simulink model "fix_all_sync"  (R2025b)
settings: Solver=FixedStepAuto  StartTime=0.0  StopTime=10.0  FixedStep=0.001  RelTol=1e-3
values from neighbouring files (symbols this model uses):
  Dm = 1e-3    (= 0.001)    [motor_param.m]
  Jm = 0.1e-3    (= 0.0001)    [motor_param.m]
  Ld = 0.01    [motor_param.m]
  Lq = 0.02    [motor_param.m]
  p = 2    [motor_param.m]
  Phi = 0.1    [motor_param.m]
  Rs = 0.38    [motor_param.m]
libraries: fl_lib x50, nesl_utility x50, ee_lib x15, eeTransforms x10, simulink x1
(part 3 of 3)

== system fix_all_sync/Subsystem5/Plant/MechSensor ==
  Ideal Rotational Motion Sensor : fl_lib/Mechanical/Mechanical Sensors/Ideal Rotational Motion Sensor  reference=foundation.enum.MeasurementReference.difference  acceleration_port=false  velocity_port=true  position_port=true  wrap_angle=simscape.enum.onoff.off  offset=0 rad
  Ideal Torque Sensor : fl_lib/Mechanical/Mechanical Sensors/Ideal Torque Sensor
  PS-Simulink Converter : nesl_utility/PS-Simulink Converter  PhysicalDomain=network_engine_domain  SubClassName=ps_output  LeftPortType=input  RightPortType=output  PseudoPeriodic=off  Frequencies=[]  VectorFormat=1-D array  Unit=1  AffineConversion=off
  PS-Simulink Converter1 : nesl_utility/PS-Simulink Converter  PhysicalDomain=network_engine_domain  SubClassName=ps_output  LeftPortType=input  RightPortType=output  PseudoPeriodic=off  Frequencies=[]  VectorFormat=1-D array  Unit=1  AffineConversion=off
  PS-Simulink Converter2 : nesl_utility/PS-Simulink Converter  PhysicalDomain=network_engine_domain  SubClassName=ps_output  LeftPortType=input  RightPortType=output  PseudoPeriodic=off  Frequencies=[]  VectorFormat=1-D array  Unit=1  AffineConversion=off
  R1 : PMIOPort  Side=Left
  C1 : PMIOPort  Port=2  Side=Left
  R2 : PMIOPort  Port=3  Side=Right
  C2 : PMIOPort  Port=4  Side=Right
  wm : Outport  VectorParamsAs1DForOutWhenUnconnected=off
  thm : Outport  Port=2  VectorParamsAs1DForOutWhenUnconnected=off
  Tm : Outport  Port=3  VectorParamsAs1DForOutWhenUnconnected=off
  wires:
  PS-Simulink Converter/1 -> thm/1
  PS-Simulink Converter1/1 -> Tm/1
  PS-Simulink Converter2/1 -> wm/1
  connections:
  Ideal Rotational Motion Sensor/RConn3 -- PS-Simulink Converter/LConn1
  Ideal Rotational Motion Sensor/RConn1 -- C2/RConn1 -- C1/RConn1
  Ideal Torque Sensor/LConn1 -- R1/RConn1
  Ideal Torque Sensor/RConn1 -- R2/RConn1 -- Ideal Rotational Motion Sensor/LConn1
  PS-Simulink Converter1/LConn1 -- Ideal Torque Sensor/RConn2
  Ideal Rotational Motion Sensor/RConn2 -- PS-Simulink Converter2/LConn1

== system fix_all_sync/Subsystem1/Controller/DriverPeripherals/Break Algebraic Loop ==
  In1 : Inport
  Demux : Demux  Outputs=3
  Mux : Mux  Inputs=3
  Transfer Fcn : TransferFcn  Denominator=[1e-6 1]
  Transfer Fcn1 : TransferFcn  Denominator=[1e-6 1]
  Transfer Fcn2 : TransferFcn  Denominator=[1e-6 1]
  Out1 : Outport
  wires:
  In1/1 -> Demux/1
  Demux/1 -> Transfer Fcn/1
  Transfer Fcn/1 -> Mux/1
  Demux/2 -> Transfer Fcn1/1
  Transfer Fcn1/1 -> Mux/2
  Demux/3 -> Transfer Fcn2/1
  Transfer Fcn2/1 -> Mux/3
  Mux/1 -> Out1/1

== system fix_all_sync/Subsystem1/Controller/FOC/CurrentController ==
  Iqref : Inport
  Id : Inport  Port=2
  Iq : Inport  Port=3
  we : Inport  Port=4
  Integrator : Integrator
  MATLAB Function : MATLAB Function  TreatAsAtomicUnit=on
  Scope : Scope
      settings: ActiveDisplayYMinimum=-0.021972241997855933  ActiveDisplayYMaximum=0.011100987286103392  DataLoggingVariableName=ScopeData15
  Vdref : Outport  VectorParamsAs1DForOutWhenUnconnected=off
  Vqref : Outport  Port=2  VectorParamsAs1DForOutWhenUnconnected=off
  wires:
  MATLAB Function/2(Vd) -> Vdref/1
  Iqref/1 -> MATLAB Function/2(i_q_ref)
  MATLAB Function/4(e_q_bar) -> Scope/1
  we/1 -> MATLAB Function/5(we)
  Id/1 -> MATLAB Function/4(i_d)
  Iq/1 -> MATLAB Function/3(i_q)
  Integrator/1 -> MATLAB Function/1(z_q)
  MATLAB Function/1(Vq) -> Vqref/1
  MATLAB Function/3(dz_q) -> Integrator/1

== system fix_all_sync/Subsystem1/Controller/FOC/VelocityController ==
  wmref : Inport
  wm : Inport  Port=2
  Gain : Gain  Gain=1/(3/2*p*Phi)
  Integrator : Integrator
  Integrator1 : Integrator
  MATLAB Function : MATLAB Function  TreatAsAtomicUnit=on
  Iqref : Outport  VectorParamsAs1DForOutWhenUnconnected=off
  wires:
  MATLAB Function/2(dot_bar_w) -> Integrator/1
  wm/1 -> MATLAB Function/2(w_m)
  MATLAB Function/1(u_cmd) -> Gain/1
  Integrator/1 -> MATLAB Function/3(bar_w)
  Gain/1 -> Iqref/1
  wmref/1 -> MATLAB Function/1(w_ref)
  MATLAB Function/3(dot_xi) -> Integrator1/1
  Integrator1/1 -> MATLAB Function/4(xi)

== system fix_all_sync/Subsystem1/Controller/FOC/abc2dq ==
  Iabc : Inport
  thetae : Inport  Port=2
  Demux1 : Demux  Outputs=3
  Park Transform : eeTransforms/Park Transform  AxisAlignment=D-axis  PowerInvariant=off
  Terminator : Terminator
  Id : Outport  VectorParamsAs1DForOutWhenUnconnected=off
  Iq : Outport  Port=2  VectorParamsAs1DForOutWhenUnconnected=off
  wires:
  Iabc/1 -> Park Transform/1
  thetae/1 -> Park Transform/2
  Demux1/3 -> Terminator/1
  Park Transform/1 -> Demux1/1
  Demux1/1 -> Id/1
  Demux1/2 -> Iq/1

== system fix_all_sync/Subsystem1/Controller/FOC/dq2abc ==
  Vd : Inport
  Vq : Inport  Port=2
  thetae : Inport  Port=3
  Constant : Constant  Value=0
  Inverse Park Transform : eeTransforms/Inverse Park Transform  AxisAlignment=D-axis  PowerInvariant=off
  Mux : Mux  Inputs=3
  Vabc : Outport  VectorParamsAs1DForOutWhenUnconnected=off
  wires:
  thetae/1 -> Inverse Park Transform/2
  Constant/1 -> Mux/3
  Mux/1 -> Inverse Park Transform/1
  Vd/1 -> Mux/1
  Inverse Park Transform/1 -> Vabc/1
  Vq/1 -> Mux/2

== system fix_all_sync/Subsystem1/Controller/FOC/thm2the ==
  thm : Inport
  Constant : Constant  Value=2*pi
  Mod : Math  Operator=mod  SignedPower=on
  PolePairs : Gain  Gain=p
  the : Outport  VectorParamsAs1DForOutWhenUnconnected=off
  wires:
  Constant/1 -> Mod/2
  PolePairs/1 -> Mod/1
  Mod/1 -> the/1
  thm/1 -> PolePairs/1

== system fix_all_sync/Subsystem1/Controller/FOC/wm2we ==
  wm : Inport
  PolePairs : Gain  Gain=p
  we : Outport  VectorParamsAs1DForOutWhenUnconnected=off
  wires:
  wm/1 -> PolePairs/1
  PolePairs/1 -> we/1

== system fix_all_sync/Subsystem2/Controller/DriverPeripherals/Break Algebraic Loop ==
  In1 : Inport
  Demux : Demux  Outputs=3
  Mux : Mux  Inputs=3
  Transfer Fcn : TransferFcn  Denominator=[1e-6 1]
  Transfer Fcn1 : TransferFcn  Denominator=[1e-6 1]
  Transfer Fcn2 : TransferFcn  Denominator=[1e-6 1]
  Out1 : Outport
  wires:
  In1/1 -> Demux/1
  Demux/1 -> Transfer Fcn/1
  Transfer Fcn/1 -> Mux/1
  Demux/2 -> Transfer Fcn1/1
  Transfer Fcn1/1 -> Mux/2
  Demux/3 -> Transfer Fcn2/1
  Transfer Fcn2/1 -> Mux/3
  Mux/1 -> Out1/1

== system fix_all_sync/Subsystem2/Controller/FOC/CurrentController ==
  Iqref : Inport
  Id : Inport  Port=2
  Iq : Inport  Port=3
  we : Inport  Port=4
  Integrator : Integrator
  MATLAB Function : MATLAB Function  TreatAsAtomicUnit=on
  Scope : Scope
      settings: ActiveDisplayYMinimum=-0.021972241997855933  ActiveDisplayYMaximum=0.011100987286103392  DataLoggingVariableName=ScopeData8
  Vdref : Outport  VectorParamsAs1DForOutWhenUnconnected=off
  Vqref : Outport  Port=2  VectorParamsAs1DForOutWhenUnconnected=off
  wires:
  Iqref/1 -> MATLAB Function/2(i_q_ref)
  MATLAB Function/4(e_q_bar) -> Scope/1
  MATLAB Function/1(Vq) -> Vqref/1
  Integrator/1 -> MATLAB Function/1(z_q)
  MATLAB Function/2(Vd) -> Vdref/1
  MATLAB Function/3(dz_q) -> Integrator/1
  Id/1 -> MATLAB Function/4(i_d)
  we/1 -> MATLAB Function/5(we)
  Iq/1 -> MATLAB Function/3(i_q)

== system fix_all_sync/Subsystem2/Controller/FOC/VelocityController ==
  wmref : Inport
  wm : Inport  Port=2
  Gain : Gain  Gain=1/(3/2*p*Phi)
  Integrator : Integrator
  Integrator1 : Integrator
  MATLAB Function : MATLAB Function  TreatAsAtomicUnit=on
  Iqref : Outport  VectorParamsAs1DForOutWhenUnconnected=off
  wires:
  Integrator/1 -> MATLAB Function/3(bar_w)
  Integrator1/1 -> MATLAB Function/4(xi)
  wmref/1 -> MATLAB Function/1(w_ref)
  MATLAB Function/3(dot_xi) -> Integrator1/1
  MATLAB Function/1(u_cmd) -> Gain/1
  Gain/1 -> Iqref/1
  wm/1 -> MATLAB Function/2(w_m)
  MATLAB Function/2(dot_bar_w) -> Integrator/1

== system fix_all_sync/Subsystem2/Controller/FOC/abc2dq ==
  Iabc : Inport
  thetae : Inport  Port=2
  Demux1 : Demux  Outputs=3
  Park Transform : eeTransforms/Park Transform  AxisAlignment=D-axis  PowerInvariant=off
  Terminator : Terminator
  Id : Outport  VectorParamsAs1DForOutWhenUnconnected=off
  Iq : Outport  Port=2  VectorParamsAs1DForOutWhenUnconnected=off
  wires:
  Iabc/1 -> Park Transform/1
  thetae/1 -> Park Transform/2
  Demux1/3 -> Terminator/1
  Park Transform/1 -> Demux1/1
  Demux1/1 -> Id/1
  Demux1/2 -> Iq/1

== system fix_all_sync/Subsystem2/Controller/FOC/dq2abc ==
  Vd : Inport
  Vq : Inport  Port=2
  thetae : Inport  Port=3
  Constant : Constant  Value=0
  Inverse Park Transform : eeTransforms/Inverse Park Transform  AxisAlignment=D-axis  PowerInvariant=off
  Mux : Mux  Inputs=3
  Vabc : Outport  VectorParamsAs1DForOutWhenUnconnected=off
  wires:
  thetae/1 -> Inverse Park Transform/2
  Constant/1 -> Mux/3
  Mux/1 -> Inverse Park Transform/1
  Vd/1 -> Mux/1
  Inverse Park Transform/1 -> Vabc/1
  Vq/1 -> Mux/2

== system fix_all_sync/Subsystem2/Controller/FOC/thm2the ==
  thm : Inport
  Constant : Constant  Value=2*pi
  Mod : Math  Operator=mod  SignedPower=on
  PolePairs : Gain  Gain=p
  the : Outport  VectorParamsAs1DForOutWhenUnconnected=off
  wires:
  Constant/1 -> Mod/2
  PolePairs/1 -> Mod/1
  Mod/1 -> the/1
  thm/1 -> PolePairs/1

== system fix_all_sync/Subsystem2/Controller/FOC/wm2we ==
  wm : Inport
  PolePairs : Gain  Gain=p
  we : Outport  VectorParamsAs1DForOutWhenUnconnected=off
  wires:
  wm/1 -> PolePairs/1
  PolePairs/1 -> we/1

== system fix_all_sync/Subsystem3/Controller/DriverPeripherals/Break Algebraic Loop ==
  In1 : Inport
  Demux : Demux  Outputs=3
  Mux : Mux  Inputs=3
  Transfer Fcn : TransferFcn  Denominator=[1e-6 1]
  Transfer Fcn1 : TransferFcn  Denominator=[1e-6 1]
  Transfer Fcn2 : TransferFcn  Denominator=[1e-6 1]
  Out1 : Outport
  wires:
  In1/1 -> Demux/1
  Demux/1 -> Transfer Fcn/1
  Transfer Fcn/1 -> Mux/1
  Demux/2 -> Transfer Fcn1/1
  Transfer Fcn1/1 -> Mux/2
  Demux/3 -> Transfer Fcn2/1
  Transfer Fcn2/1 -> Mux/3
  Mux/1 -> Out1/1

== system fix_all_sync/Subsystem3/Controller/FOC/CurrentController ==
  Iqref : Inport
  Id : Inport  Port=2
  Iq : Inport  Port=3
  we : Inport  Port=4
  Integrator : Integrator
  MATLAB Function : MATLAB Function  TreatAsAtomicUnit=on
  Scope : Scope
      settings: ActiveDisplayYMinimum=-0.021972241997855933  ActiveDisplayYMaximum=0.011100987286103392  DataLoggingVariableName=ScopeData9
  Vdref : Outport  VectorParamsAs1DForOutWhenUnconnected=off
  Vqref : Outport  Port=2  VectorParamsAs1DForOutWhenUnconnected=off
  wires:
  Iqref/1 -> MATLAB Function/2(i_q_ref)
  MATLAB Function/4(e_q_bar) -> Scope/1
  MATLAB Function/1(Vq) -> Vqref/1
  Integrator/1 -> MATLAB Function/1(z_q)
  MATLAB Function/2(Vd) -> Vdref/1
  MATLAB Function/3(dz_q) -> Integrator/1
  Id/1 -> MATLAB Function/4(i_d)
  Iq/1 -> MATLAB Function/3(i_q)
  we/1 -> MATLAB Function/5(we)

== system fix_all_sync/Subsystem3/Controller/FOC/VelocityController ==
  wmref : Inport
  wm : Inport  Port=2
  Gain : Gain  Gain=1/(3/2*p*Phi)
  Integrator : Integrator
  Integrator1 : Integrator
  MATLAB Function : MATLAB Function  TreatAsAtomicUnit=on
  Iqref : Outport  VectorParamsAs1DForOutWhenUnconnected=off
  wires:
  Integrator/1 -> MATLAB Function/3(bar_w)
  Integrator1/1 -> MATLAB Function/4(xi)
  wmref/1 -> MATLAB Function/1(w_ref)
  MATLAB Function/3(dot_xi) -> Integrator1/1
  MATLAB Function/1(u_cmd) -> Gain/1
  Gain/1 -> Iqref/1
  wm/1 -> MATLAB Function/2(w_m)
  MATLAB Function/2(dot_bar_w) -> Integrator/1

== system fix_all_sync/Subsystem3/Controller/FOC/abc2dq ==
  Iabc : Inport
  thetae : Inport  Port=2
  Demux1 : Demux  Outputs=3
  Park Transform : eeTransforms/Park Transform  AxisAlignment=D-axis  PowerInvariant=off
  Terminator : Terminator
  Id : Outport  VectorParamsAs1DForOutWhenUnconnected=off
  Iq : Outport  Port=2  VectorParamsAs1DForOutWhenUnconnected=off
  wires:
  Iabc/1 -> Park Transform/1
  thetae/1 -> Park Transform/2
  Demux1/3 -> Terminator/1
  Park Transform/1 -> Demux1/1
  Demux1/1 -> Id/1
  Demux1/2 -> Iq/1

== system fix_all_sync/Subsystem3/Controller/FOC/dq2abc ==
  Vd : Inport
  Vq : Inport  Port=2
  thetae : Inport  Port=3
  Constant : Constant  Value=0
  Inverse Park Transform : eeTransforms/Inverse Park Transform  AxisAlignment=D-axis  PowerInvariant=off
  Mux : Mux  Inputs=3
  Vabc : Outport  VectorParamsAs1DForOutWhenUnconnected=off
  wires:
  thetae/1 -> Inverse Park Transform/2
  Constant/1 -> Mux/3
  Mux/1 -> Inverse Park Transform/1
  Vd/1 -> Mux/1
  Inverse Park Transform/1 -> Vabc/1
  Vq/1 -> Mux/2

== system fix_all_sync/Subsystem3/Controller/FOC/thm2the ==
  thm : Inport
  Constant : Constant  Value=2*pi
  Mod : Math  Operator=mod  SignedPower=on
  PolePairs : Gain  Gain=p
  the : Outport  VectorParamsAs1DForOutWhenUnconnected=off
  wires:
  Constant/1 -> Mod/2
  PolePairs/1 -> Mod/1
  Mod/1 -> the/1
  thm/1 -> PolePairs/1

== system fix_all_sync/Subsystem3/Controller/FOC/wm2we ==
  wm : Inport
  PolePairs : Gain  Gain=p
  we : Outport  VectorParamsAs1DForOutWhenUnconnected=off
  wires:
  wm/1 -> PolePairs/1
  PolePairs/1 -> we/1

== system fix_all_sync/Subsystem4/Controller/DriverPeripherals/Break Algebraic Loop ==
  In1 : Inport
  Demux : Demux  Outputs=3
  Mux : Mux  Inputs=3
  Transfer Fcn : TransferFcn  Denominator=[1e-6 1]
  Transfer Fcn1 : TransferFcn  Denominator=[1e-6 1]
  Transfer Fcn2 : TransferFcn  Denominator=[1e-6 1]
  Out1 : Outport
  wires:
  In1/1 -> Demux/1
  Demux/1 -> Transfer Fcn/1
  Transfer Fcn/1 -> Mux/1
  Demux/2 -> Transfer Fcn1/1
  Transfer Fcn1/1 -> Mux/2
  Demux/3 -> Transfer Fcn2/1
  Transfer Fcn2/1 -> Mux/3
  Mux/1 -> Out1/1

== system fix_all_sync/Subsystem4/Controller/FOC/CurrentController ==
  Iqref : Inport
  Id : Inport  Port=2
  Iq : Inport  Port=3
  we : Inport  Port=4
  Integrator : Integrator
  MATLAB Function : MATLAB Function  TreatAsAtomicUnit=on
  Scope : Scope
      settings: ActiveDisplayYMinimum=-0.021972241997855933  ActiveDisplayYMaximum=0.011100987286103392  DataLoggingVariableName=ScopeData10
  Vdref : Outport  VectorParamsAs1DForOutWhenUnconnected=off
  Vqref : Outport  Port=2  VectorParamsAs1DForOutWhenUnconnected=off
  wires:
  Iqref/1 -> MATLAB Function/2(i_q_ref)
  MATLAB Function/4(e_q_bar) -> Scope/1
  MATLAB Function/1(Vq) -> Vqref/1
  Integrator/1 -> MATLAB Function/1(z_q)
  MATLAB Function/2(Vd) -> Vdref/1
  MATLAB Function/3(dz_q) -> Integrator/1
  Id/1 -> MATLAB Function/4(i_d)
  Iq/1 -> MATLAB Function/3(i_q)
  we/1 -> MATLAB Function/5(we)

== system fix_all_sync/Subsystem4/Controller/FOC/VelocityController ==
  wmref : Inport
  wm : Inport  Port=2
  Gain : Gain  Gain=1/(3/2*p*Phi)
  Integrator : Integrator
  Integrator1 : Integrator
  MATLAB Function : MATLAB Function  TreatAsAtomicUnit=on
  Iqref : Outport  VectorParamsAs1DForOutWhenUnconnected=off
  wires:
  Integrator/1 -> MATLAB Function/3(bar_w)
  Integrator1/1 -> MATLAB Function/4(xi)
  wmref/1 -> MATLAB Function/1(w_ref)
  MATLAB Function/3(dot_xi) -> Integrator1/1
  MATLAB Function/1(u_cmd) -> Gain/1
  Gain/1 -> Iqref/1
  wm/1 -> MATLAB Function/2(w_m)
  MATLAB Function/2(dot_bar_w) -> Integrator/1

== system fix_all_sync/Subsystem4/Controller/FOC/abc2dq ==
  Iabc : Inport
  thetae : Inport  Port=2
  Demux1 : Demux  Outputs=3
  Park Transform : eeTransforms/Park Transform  AxisAlignment=D-axis  PowerInvariant=off
  Terminator : Terminator
  Id : Outport  VectorParamsAs1DForOutWhenUnconnected=off
  Iq : Outport  Port=2  VectorParamsAs1DForOutWhenUnconnected=off
  wires:
  Iabc/1 -> Park Transform/1
  thetae/1 -> Park Transform/2
  Demux1/3 -> Terminator/1
  Park Transform/1 -> Demux1/1
  Demux1/1 -> Id/1
  Demux1/2 -> Iq/1

== system fix_all_sync/Subsystem4/Controller/FOC/dq2abc ==
  Vd : Inport
  Vq : Inport  Port=2
  thetae : Inport  Port=3
  Constant : Constant  Value=0
  Inverse Park Transform : eeTransforms/Inverse Park Transform  AxisAlignment=D-axis  PowerInvariant=off
  Mux : Mux  Inputs=3
  Vabc : Outport  VectorParamsAs1DForOutWhenUnconnected=off
  wires:
  thetae/1 -> Inverse Park Transform/2
  Constant/1 -> Mux/3
  Mux/1 -> Inverse Park Transform/1
  Vd/1 -> Mux/1
  Inverse Park Transform/1 -> Vabc/1
  Vq/1 -> Mux/2

== system fix_all_sync/Subsystem4/Controller/FOC/thm2the ==
  thm : Inport
  Constant : Constant  Value=2*pi
  Mod : Math  Operator=mod  SignedPower=on
  PolePairs : Gain  Gain=p
  the : Outport  VectorParamsAs1DForOutWhenUnconnected=off
  wires:
  Constant/1 -> Mod/2
  PolePairs/1 -> Mod/1
  Mod/1 -> the/1
  thm/1 -> PolePairs/1

== system fix_all_sync/Subsystem4/Controller/FOC/wm2we ==
  wm : Inport
  PolePairs : Gain  Gain=p
  we : Outport  VectorParamsAs1DForOutWhenUnconnected=off
  wires:
  wm/1 -> PolePairs/1
  PolePairs/1 -> we/1

== system fix_all_sync/Subsystem5/Controller/DriverPeripherals/Break Algebraic Loop ==
  In1 : Inport
  Demux : Demux  Outputs=3
  Mux : Mux  Inputs=3
  Transfer Fcn : TransferFcn  Denominator=[1e-6 1]
  Transfer Fcn1 : TransferFcn  Denominator=[1e-6 1]
  Transfer Fcn2 : TransferFcn  Denominator=[1e-6 1]
  Out1 : Outport
  wires:
  In1/1 -> Demux/1
  Demux/1 -> Transfer Fcn/1
  Transfer Fcn/1 -> Mux/1
  Demux/2 -> Transfer Fcn1/1
  Transfer Fcn1/1 -> Mux/2
  Demux/3 -> Transfer Fcn2/1
  Transfer Fcn2/1 -> Mux/3
  Mux/1 -> Out1/1

== system fix_all_sync/Subsystem5/Controller/FOC/CurrentController ==
  Iqref : Inport
  Id : Inport  Port=2
  Iq : Inport  Port=3
  we : Inport  Port=4
  Integrator : Integrator
  MATLAB Function : MATLAB Function  TreatAsAtomicUnit=on
  Scope : Scope
      settings: ActiveDisplayYMinimum=-0.021972241997855933  ActiveDisplayYMaximum=0.011100987286103392  DataLoggingVariableName=ScopeData11
  Vdref : Outport  VectorParamsAs1DForOutWhenUnconnected=off
  Vqref : Outport  Port=2  VectorParamsAs1DForOutWhenUnconnected=off
  wires:
  Iqref/1 -> MATLAB Function/2(i_q_ref)
  MATLAB Function/4(e_q_bar) -> Scope/1
  MATLAB Function/1(Vq) -> Vqref/1
  Integrator/1 -> MATLAB Function/1(z_q)
  MATLAB Function/2(Vd) -> Vdref/1
  MATLAB Function/3(dz_q) -> Integrator/1
  Id/1 -> MATLAB Function/4(i_d)
  Iq/1 -> MATLAB Function/3(i_q)
  we/1 -> MATLAB Function/5(we)

== system fix_all_sync/Subsystem5/Controller/FOC/VelocityController ==
  wmref : Inport
  wm : Inport  Port=2
  Gain : Gain  Gain=1/(3/2*p*Phi)
  Integrator : Integrator
  Integrator1 : Integrator
  MATLAB Function : MATLAB Function  TreatAsAtomicUnit=on
  Iqref : Outport  VectorParamsAs1DForOutWhenUnconnected=off
  wires:
  Integrator/1 -> MATLAB Function/3(bar_w)
  Integrator1/1 -> MATLAB Function/4(xi)
  wmref/1 -> MATLAB Function/1(w_ref)
  MATLAB Function/3(dot_xi) -> Integrator1/1
  MATLAB Function/1(u_cmd) -> Gain/1
  Gain/1 -> Iqref/1
  wm/1 -> MATLAB Function/2(w_m)
  MATLAB Function/2(dot_bar_w) -> Integrator/1

== system fix_all_sync/Subsystem5/Controller/FOC/abc2dq ==
  Iabc : Inport
  thetae : Inport  Port=2
  Demux1 : Demux  Outputs=3
  Park Transform : eeTransforms/Park Transform  AxisAlignment=D-axis  PowerInvariant=off
  Terminator : Terminator
  Id : Outport  VectorParamsAs1DForOutWhenUnconnected=off
  Iq : Outport  Port=2  VectorParamsAs1DForOutWhenUnconnected=off
  wires:
  Iabc/1 -> Park Transform/1
  thetae/1 -> Park Transform/2
  Demux1/3 -> Terminator/1
  Park Transform/1 -> Demux1/1
  Demux1/1 -> Id/1
  Demux1/2 -> Iq/1

== system fix_all_sync/Subsystem5/Controller/FOC/dq2abc ==
  Vd : Inport
  Vq : Inport  Port=2
  thetae : Inport  Port=3
  Constant : Constant  Value=0
  Inverse Park Transform : eeTransforms/Inverse Park Transform  AxisAlignment=D-axis  PowerInvariant=off
  Mux : Mux  Inputs=3
  Vabc : Outport  VectorParamsAs1DForOutWhenUnconnected=off
  wires:
  thetae/1 -> Inverse Park Transform/2
  Constant/1 -> Mux/3
  Mux/1 -> Inverse Park Transform/1
  Vd/1 -> Mux/1
  Inverse Park Transform/1 -> Vabc/1
  Vq/1 -> Mux/2

== system fix_all_sync/Subsystem5/Controller/FOC/thm2the ==
  thm : Inport
  Constant : Constant  Value=2*pi
  Mod : Math  Operator=mod  SignedPower=on
  PolePairs : Gain  Gain=p
  the : Outport  VectorParamsAs1DForOutWhenUnconnected=off
  wires:
  Constant/1 -> Mod/2
  PolePairs/1 -> Mod/1
  Mod/1 -> the/1
  thm/1 -> PolePairs/1

== system fix_all_sync/Subsystem5/Controller/FOC/wm2we ==
  wm : Inport
  PolePairs : Gain  Gain=p
  we : Outport  VectorParamsAs1DForOutWhenUnconnected=off
  wires:
  wm/1 -> PolePairs/1
  PolePairs/1 -> we/1

== matlab function fix_all_sync/Subsystem2/Controller/FOC/VelocityController/MATLAB Function ==
  data: w_ref input; u_cmd output; w_m input; bar_w input; xi input; Jm parameter; Dm parameter; dot_bar_w output; dot_xi output
function [u_cmd, dot_bar_w, dot_xi] = FixedTimeController(w_ref, w_m, bar_w, xi, Jm, Dm)

    lambda1  = 5;   lambda2 = 5;   lambda3 = 6;
    tau      = 0.5; vartheta = 1.5;
    k_w = 6; k1 = 5; k2 = 5;

    k_i = 20;

    kappa0 = 30;     % 线性积分增益（新增，压制小误差）
    kappa1 = 20;     % 固定时间项增益
    kappa2 = 20;
    alpha1 = 0.5;
    alpha2 = 1.5;

    pow_func = @(x, gamma) abs(x)^gamma * sign(x);

    % 公式(117) 滤波器
    e_w = bar_w - w_ref;
    dot_bar_w = (1/tau) * ( -lambda1 * pow_func(e_w, 0.5) ...
                            -lambda2 * pow_func(e_w, vartheta) ...
                            -lambda3 * e_w );

    s   = w_m - bar_w;
    e_v = w_m - w_ref;

    % 混合固定时间积分
    dot_xi = kappa0 * e_v ...
           + kappa1 * pow_func(e_v, alpha1) ...
           + kappa2 * pow_func(e_v, alpha2);

    TL_hat_int = k_i * xi;

    feedback = -k_w * s ...
               - k1 * pow_func(s, 0.5) ...
               - k2 * pow_func(s, vartheta);

    u_cmd = Jm * dot_bar_w + Dm * bar_w - TL_hat_int + feedback;
end

== matlab function fix_all_sync/Subsystem3/Controller/FOC/VelocityController/MATLAB Function ==
  data: w_ref input; u_cmd output; w_m input; bar_w input; xi input; Jm parameter; Dm parameter; dot_bar_w output; dot_xi output
function [u_cmd, dot_bar_w, dot_xi] = FixedTimeController(w_ref, w_m, bar_w, xi, Jm, Dm)

    lambda1  = 5;   lambda2 = 5;   lambda3 = 6;
    tau      = 0.5; vartheta = 1.5;
    k_w = 6; k1 = 5; k2 = 5;

    k_i = 20;

    kappa0 = 30;     % 线性积分增益（新增，压制小误差）
    kappa1 = 20;     % 固定时间项增益
    kappa2 = 20;
    alpha1 = 0.5;
    alpha2 = 1.5;

    pow_func = @(x, gamma) abs(x)^gamma * sign(x);

    % 公式(117) 滤波器
    e_w = bar_w - w_ref;
    dot_bar_w = (1/tau) * ( -lambda1 * pow_func(e_w, 0.5) ...
                            -lambda2 * pow_func(e_w, vartheta) ...
                            -lambda3 * e_w );

    s   = w_m - bar_w;
    e_v = w_m - w_ref;

    % 混合固定时间积分
    dot_xi = kappa0 * e_v ...
           + kappa1 * pow_func(e_v, alpha1) ...
           + kappa2 * pow_func(e_v, alpha2);

    TL_hat_int = k_i * xi;

    feedback = -k_w * s ...
               - k1 * pow_func(s, 0.5) ...
               - k2 * pow_func(s, vartheta);

    u_cmd = Jm * dot_bar_w + Dm * bar_w - TL_hat_int + feedback;
end

== matlab function fix_all_sync/Subsystem4/Controller/FOC/VelocityController/MATLAB Function ==
  data: w_ref input; u_cmd output; w_m input; bar_w input; xi input; Jm parameter; Dm parameter; dot_bar_w output; dot_xi output
function [u_cmd, dot_bar_w, dot_xi] = FixedTimeController(w_ref, w_m, bar_w, xi, Jm, Dm)

    lambda1  = 5;   lambda2 = 5;   lambda3 = 6;
    tau      = 0.5; vartheta = 1.5;
    k_w = 6; k1 = 5; k2 = 5;

    k_i = 20;

    kappa0 = 30;     % 线性积分增益（新增，压制小误差）
    kappa1 = 20;     % 固定时间项增益
    kappa2 = 20;
    alpha1 = 0.5;
    alpha2 = 1.5;

    pow_func = @(x, gamma) abs(x)^gamma * sign(x);

    % 公式(117) 滤波器
    e_w = bar_w - w_ref;
    dot_bar_w = (1/tau) * ( -lambda1 * pow_func(e_w, 0.5) ...
                            -lambda2 * pow_func(e_w, vartheta) ...
                            -lambda3 * e_w );

    s   = w_m - bar_w;
    e_v = w_m - w_ref;

    % 混合固定时间积分
    dot_xi = kappa0 * e_v ...
           + kappa1 * pow_func(e_v, alpha1) ...
           + kappa2 * pow_func(e_v, alpha2);

    TL_hat_int = k_i * xi;

    feedback = -k_w * s ...
               - k1 * pow_func(s, 0.5) ...
               - k2 * pow_func(s, vartheta);

    u_cmd = Jm * dot_bar_w + Dm * bar_w - TL_hat_int + feedback;
end

== matlab function fix_all_sync/Subsystem5/Controller/FOC/VelocityController/MATLAB Function ==
  data: w_ref input; u_cmd output; w_m input; bar_w input; xi input; Jm parameter; Dm parameter; dot_bar_w output; dot_xi output
function [u_cmd, dot_bar_w, dot_xi] = FixedTimeController(w_ref, w_m, bar_w, xi, Jm, Dm)

    lambda1  = 5;   lambda2 = 5;   lambda3 = 6;
    tau      = 0.5; vartheta = 1.5;
    k_w = 6; k1 = 5; k2 = 5;

    k_i = 20;

    kappa0 = 30;     % 线性积分增益（新增，压制小误差）
    kappa1 = 20;     % 固定时间项增益
    kappa2 = 20;
    alpha1 = 0.5;
    alpha2 = 1.5;

    pow_func = @(x, gamma) abs(x)^gamma * sign(x);

    % 公式(117) 滤波器
    e_w = bar_w - w_ref;
    dot_bar_w = (1/tau) * ( -lambda1 * pow_func(e_w, 0.5) ...
                            -lambda2 * pow_func(e_w, vartheta) ...
                            -lambda3 * e_w );

    s   = w_m - bar_w;
    e_v = w_m - w_ref;

    % 混合固定时间积分
    dot_xi = kappa0 * e_v ...
           + kappa1 * pow_func(e_v, alpha1) ...
           + kappa2 * pow_func(e_v, alpha2);

    TL_hat_int = k_i * xi;

    feedback = -k_w * s ...
               - k1 * pow_func(s, 0.5) ...
               - k2 * pow_func(s, vartheta);

    u_cmd = Jm * dot_bar_w + Dm * bar_w - TL_hat_int + feedback;
end

== matlab function fix_all_sync/Subsystem7/MATLAB Function4 ==
  data: dth_hat output; dom_hat output; theta0 input; th_hat input; om_hat input
%% ObserverRHS
function [dth_hat, dom_hat] = ObserverRHS(theta0, th_hat, om_hat)
%#codegen
n = 5;
L = 2*eye(n) - diag(ones(n-1,1),1) - diag(ones(n-1,1),-1);
B = diag([1, 0, 1, 0, 0]);

a1 = 0.7;  a2 = 1.3;
a3 = 2*a1-1;  a4 = 2*a2-1;
c1 = 50;  c2 = 50;     % ★ 加大
c3 = 500; c4 = 500;    % ★ 加大

sig = @(x,a) sign(x).*abs(x).^a;

th0 = theta0(1);       % ★ 强制标量

e = zeros(n,1);
for i = 1:n
    ei = 0;
    for j = 1:n
        if i ~= j && L(i,j) ~= 0
            ei = ei + (-L(i,j))*(th_hat(i) - th_hat(j));
        end
    end
    if B(i,i) == 1
        ei = ei + (th_hat(i) - th0);
    end
    e(i) = ei;
end

dth_hat = om_hat - c1*sig(e,a1) - c2*sig(e,a2);
dom_hat =          - c3*sig(e,a3) - c4*sig(e,a4);
end

== matlab function fix_all_sync/Subsystem1/Controller/FOC/CurrentController/MATLAB Function ==
  data: z_q input; Vq output; i_q_ref input; i_q input; i_d input; we input; Vd output; dz_q output; e_q_bar output; Rs parameter; Ld parameter; Lq parameter; Phi parameter
function [Vq, Vd, dz_q, e_q_bar] = smc_ctrl(z_q, i_q_ref, i_q, i_d, we, Rs, Ld, Lq, Phi)
%#codegen
% ============================================================
%  PMSM 超螺旋滑模电流控制器
%  Rs, Ld, Lq, Phi, p 及滑模增益均由 Parameter 作用域提供
% ============================================================

%% ---------- 滑模参数 (仍然写死, 因为它们只属于控制器) ----------
r1  = 0.5;   r2  = 1.5;
rho1 = 0.5;  rho2 = 1.5;

k_q1 = -500;  k_q2 = -400;
k_d1 = -500;  k_d2 = -400;

lam_q1 = 50;   lam_q2 = 50;

%% ---------- 滑模面 ----------
e_q_bar = i_q - z_q;

%% ---------- 迭代部分的导数 (积分交给 Simulink) ----------
e_z  = z_q - i_q_ref;
dz_q = -lam_q1 * sig(e_z, rho1) - lam_q2 * sig(e_z, rho2);

%% ---------- u_q (非迭代) ----------
Vq = Lq * ( dz_q ...
             + k_q1 * sig(e_q_bar, r1) ...
             + k_q2 * sig(e_q_bar, r2) ) ...
      + Rs * z_q ...
      + Ld * we * i_d ...
      + we * Phi ;

%% ---------- u_d (非迭代) ----------
Vd = Ld * ( k_d1 * sig(i_d, r1) ...
             + k_d2 * sig(i_d, r2) ) ...
      + Rs * i_d ...
      + Lq * we * i_q;

end

function y = sig(x, r)
    y = abs(x)^r * sign(x);
end

== matlab function fix_all_sync/Subsystem1/Controller/FOC/VelocityController/MATLAB Function ==
  data: w_ref input; u_cmd output; w_m input; bar_w input; xi input; Jm parameter; Dm parameter; dot_bar_w output; dot_xi output
function [u_cmd, dot_bar_w, dot_xi] = FixedTimeController(w_ref, w_m, bar_w, xi, Jm, Dm)

    lambda1  = 5;   lambda2 = 5;   lambda3 = 6;
    tau      = 0.5; vartheta = 1.5;
    k_w = 6; k1 = 5; k2 = 5;

    k_i = 20;

    kappa0 = 30;     % 线性积分增益（新增，压制小误差）
    kappa1 = 20;     % 固定时间项增益
    kappa2 = 20;
    alpha1 = 0.5;
    alpha2 = 1.5;

    pow_func = @(x, gamma) abs(x)^gamma * sign(x);

    % 公式(117) 滤波器
    e_w = bar_w - w_ref;
    dot_bar_w = (1/tau) * ( -lambda1 * pow_func(e_w, 0.5) ...
                            -lambda2 * pow_func(e_w, vartheta) ...
                            -lambda3 * e_w );

    s   = w_m - bar_w;
    e_v = w_m - w_ref;

    % 混合固定时间积分
    dot_xi = kappa0 * e_v ...
           + kappa1 * pow_func(e_v, alpha1) ...
           + kappa2 * pow_func(e_v, alpha2);

    TL_hat_int = k_i * xi;

    feedback = -k_w * s ...
               - k1 * pow_func(s, 0.5) ...
               - k2 * pow_func(s, vartheta);

    u_cmd = Jm * dot_bar_w + Dm * bar_w - TL_hat_int + feedback;
end

== matlab function fix_all_sync/Subsystem7/MATLAB Function ==
  data: theta0 input; omega_cmd output; theta_meas input; om_hat input
function omega_cmd  = Controller(theta0, theta_meas, om_hat)
%#codegen
% 输入:
%   theta0     - 领导者角度（标量）
%   theta_meas - 5x1 电机角度（编码器）
%   om_hat     - 5x1 前馈（观测器估计的领导者角速度）
%   v_f        - 5x1 低通滤波状态（来自 Integrator）
% 输出:
%   omega_cmd  - 5x1 未滤波控制器输出（仅记录/监控）
%   dv_f       - 5x1 滤波状态导数（送 Integrator）

n = 5;
L = 2*eye(n) - diag(ones(n-1,1),1) - diag(ones(n-1,1),-1);
B = diag([1, 0, 1, 0, 0]);

p1 = 0.75;  p2 = 1.5;
k1 = 5;    k2 = 5;

tau_f = 1e-2;   % ★ 低通时间常数

sig = @(x,a) sign(x).*abs(x).^a;
th0 = theta0(1);   % 强制标量

omega_cmd = zeros(n,1);
for i = 1:n
    ei = 0;
    for j = 1:n
        if i ~= j && L(i,j) ~= 0
            ei = ei + (-L(i,j))*(theta_meas(i) - theta_meas(j));
        end
    end
    if B(i,i) == 1
        ei = ei + (theta_meas(i) - th0);
    end
    omega_cmd(i) = min(max(om_hat(i) - k1*sig(ei,p1) - k2*sig(ei,p2),-50),50);
end


end

== matlab function fix_all_sync/Subsystem2/Controller/FOC/CurrentController/MATLAB Function ==
  data: z_q input; Vq output; i_q_ref input; i_q input; i_d input; we input; Vd output; dz_q output; e_q_bar output; Rs parameter; Ld parameter; Lq parameter; Phi parameter
function [Vq, Vd, dz_q, e_q_bar] = smc_ctrl(z_q, i_q_ref, i_q, i_d, we, Rs, Ld, Lq, Phi)
%#codegen
% ============================================================
%  PMSM 超螺旋滑模电流控制器
%  Rs, Ld, Lq, Phi, p 及滑模增益均由 Parameter 作用域提供
% ============================================================

%% ---------- 滑模参数 (仍然写死, 因为它们只属于控制器) ----------
r1  = 0.5;   r2  = 1.5;
rho1 = 0.5;  rho2 = 1.5;

k_q1 = -500;  k_q2 = -400;
k_d1 = -500;  k_d2 = -400;

lam_q1 = 50;   lam_q2 = 50;

%% ---------- 滑模面 ----------
e_q_bar = i_q - z_q;

%% ---------- 迭代部分的导数 (积分交给 Simulink) ----------
e_z  = z_q - i_q_ref;
dz_q = -lam_q1 * sig(e_z, rho1) - lam_q2 * sig(e_z, rho2);

%% ---------- u_q (非迭代) ----------
Vq = Lq * ( dz_q ...
             + k_q1 * sig(e_q_bar, r1) ...
             + k_q2 * sig(e_q_bar, r2) ) ...
      + Rs * z_q ...
      + Ld * we * i_d ...
      + we * Phi ;

%% ---------- u_d (非迭代) ----------
Vd = Ld * ( k_d1 * sig(i_d, r1) ...
             + k_d2 * sig(i_d, r2) ) ...
      + Rs * i_d ...
      + Lq * we * i_q;

end

function y = sig(x, r)
    y = abs(x)^r * sign(x);
end

== matlab function fix_all_sync/Subsystem3/Controller/FOC/CurrentController/MATLAB Function ==
  data: z_q input; Vq output; i_q_ref input; i_q input; i_d input; we input; Vd output; dz_q output; e_q_bar output; Rs parameter; Ld parameter; Lq parameter; Phi parameter
function [Vq, Vd, dz_q, e_q_bar] = smc_ctrl(z_q, i_q_ref, i_q, i_d, we, Rs, Ld, Lq, Phi)
%#codegen
% ============================================================
%  PMSM 超螺旋滑模电流控制器
%  Rs, Ld, Lq, Phi, p 及滑模增益均由 Parameter 作用域提供
% ============================================================

%% ---------- 滑模参数 (仍然写死, 因为它们只属于控制器) ----------
r1  = 0.5;   r2  = 1.5;
rho1 = 0.5;  rho2 = 1.5;

k_q1 = -500;  k_q2 = -400;
k_d1 = -500;  k_d2 = -400;

lam_q1 = 50;   lam_q2 = 50;

%% ---------- 滑模面 ----------
e_q_bar = i_q - z_q;

%% ---------- 迭代部分的导数 (积分交给 Simulink) ----------
e_z  = z_q - i_q_ref;
dz_q = -lam_q1 * sig(e_z, rho1) - lam_q2 * sig(e_z, rho2);

%% ---------- u_q (非迭代) ----------
Vq = Lq * ( dz_q ...
             + k_q1 * sig(e_q_bar, r1) ...
             + k_q2 * sig(e_q_bar, r2) ) ...
      + Rs * z_q ...
      + Ld * we * i_d ...
      + we * Phi ;

%% ---------- u_d (非迭代) ----------
Vd = Ld * ( k_d1 * sig(i_d, r1) ...
             + k_d2 * sig(i_d, r2) ) ...
      + Rs * i_d ...
      + Lq * we * i_q;

end

function y = sig(x, r)
    y = abs(x)^r * sign(x);
end

== matlab function fix_all_sync/Subsystem4/Controller/FOC/CurrentController/MATLAB Function ==
  data: z_q input; Vq output; i_q_ref input; i_q input; i_d input; we input; Vd output; dz_q output; e_q_bar output; Rs parameter; Ld parameter; Lq parameter; Phi parameter
function [Vq, Vd, dz_q, e_q_bar] = smc_ctrl(z_q, i_q_ref, i_q, i_d, we, Rs, Ld, Lq, Phi)
%#codegen
% ============================================================
%  PMSM 超螺旋滑模电流控制器
%  Rs, Ld, Lq, Phi, p 及滑模增益均由 Parameter 作用域提供
% ============================================================

%% ---------- 滑模参数 (仍然写死, 因为它们只属于控制器) ----------
r1  = 0.5;   r2  = 1.5;
rho1 = 0.5;  rho2 = 1.5;

k_q1 = -500;  k_q2 = -400;
k_d1 = -500;  k_d2 = -400;

lam_q1 = 50;   lam_q2 = 50;

%% ---------- 滑模面 ----------
e_q_bar = i_q - z_q;

%% ---------- 迭代部分的导数 (积分交给 Simulink) ----------
e_z  = z_q - i_q_ref;
dz_q = -lam_q1 * sig(e_z, rho1) - lam_q2 * sig(e_z, rho2);

%% ---------- u_q (非迭代) ----------
Vq = Lq * ( dz_q ...
             + k_q1 * sig(e_q_bar, r1) ...
             + k_q2 * sig(e_q_bar, r2) ) ...
      + Rs * z_q ...
      + Ld * we * i_d ...
      + we * Phi ;

%% ---------- u_d (非迭代) ----------
Vd = Ld * ( k_d1 * sig(i_d, r1) ...
             + k_d2 * sig(i_d, r2) ) ...
      + Rs * i_d ...
      + Lq * we * i_q;

end

function y = sig(x, r)
    y = abs(x)^r * sign(x);
end

== matlab function fix_all_sync/Subsystem5/Controller/FOC/CurrentController/MATLAB Function ==
  data: z_q input; Vq output; i_q_ref input; i_q input; i_d input; we input; Vd output; dz_q output; e_q_bar output; Rs parameter; Ld parameter; Lq parameter; Phi parameter
function [Vq, Vd, dz_q, e_q_bar] = smc_ctrl(z_q, i_q_ref, i_q, i_d, we, Rs, Ld, Lq, Phi)
%#codegen
% ============================================================
%  PMSM 超螺旋滑模电流控制器
%  Rs, Ld, Lq, Phi, p 及滑模增益均由 Parameter 作用域提供
% ============================================================

%% ---------- 滑模参数 (仍然写死, 因为它们只属于控制器) ----------
r1  = 0.5;   r2  = 1.5;
rho1 = 0.5;  rho2 = 1.5;

k_q1 = -500;  k_q2 = -400;
k_d1 = -500;  k_d2 = -400;

lam_q1 = 50;   lam_q2 = 50;

%% ---------- 滑模面 ----------
e_q_bar = i_q - z_q;

%% ---------- 迭代部分的导数 (积分交给 Simulink) ----------
e_z  = z_q - i_q_ref;
dz_q = -lam_q1 * sig(e_z, rho1) - lam_q2 * sig(e_z, rho2);

%% ---------- u_q (非迭代) ----------
Vq = Lq * ( dz_q ...
             + k_q1 * sig(e_q_bar, r1) ...
             + k_q2 * sig(e_q_bar, r2) ) ...
      + Rs * z_q ...
      + Ld * we * i_d ...
      + we * Phi ;

%% ---------- u_d (非迭代) ----------
Vd = Ld * ( k_d1 * sig(i_d, r1) ...
             + k_d2 * sig(i_d, r2) ) ...
      + Rs * i_d ...
      + Lq * we * i_q;

end

function y = sig(x, r)
    y = abs(x)^r * sign(x);
end
